simulink model "extra_tip_sim"  (Simulink 9.0)
settings: Solver=FixedStepDiscrete  StartTime=start_time  StopTime=stop_time  FixedStep=0.020  RelTol=1e-3  EnableMultiTasking=on
InitFcn:
  | extra_tip_sim_init
values from neighbouring files (symbols this model uses):
  bucketAngle = WeighDebug_TOAbucket_angle_t27    [extra_tip_sim_init.m]
  imuX = WeighDebug_TOAeef_imu_accelX_t27    [extra_tip_sim_init.m]    (also in imu_pitch_cal_sim_init.m = WeighDebug_TOAeef_imu_accelX_t194)
  imuY = WeighDebug_TOAeef_imu_accelY_t27    [extra_tip_sim_init.m]    (also in imu_pitch_cal_sim_init.m = WeighDebug_TOAeef_imu_accelY_t194)
  imuZ = WeighDebug_TOAeef_imu_accelZ_t27    [extra_tip_sim_init.m]    (also in imu_pitch_cal_sim_init.m = WeighDebug_TOAeef_imu_accelZ_t194)
  liftAngle = WeighDebug_TOAlift_angle_t27    [extra_tip_sim_init.m]    (also in imu_pitch_cal_sim_init.m = WeighDebug_TOAlift_angle_t194)
  liftCmd = WeighDebug_TOAlift_valve_cmd_t27    [extra_tip_sim_init.m]
  liftCylLength = WeighDebug_LiftCylNormLen_t27    [extra_tip_sim_init.m]    (also in imu_pitch_cal_sim_init.m = WeighDebug_LiftCylLenghtNorm_Val_t194)
  liftCylPress = WeighDebug_LiftCylPres_t27    [extra_tip_sim_init.m]    (also in imu_pitch_cal_sim_init.m = WeighDebug_LiftCylPres_t194)
  payloadTarget = TOAtestPts_toa_payload_target_final_t27    [extra_tip_sim_init.m]
  steerAng = WeighDebug_TOAsteering_angle_t27    [extra_tip_sim_init.m]    (also in imu_pitch_cal_sim_init.m = WeighDebug_TOAsteering_angle_t194)
  tiltCmd = WeighDebug_TOAtilt_valve_cmd_t27    [extra_tip_sim_init.m]
  tiltExt = WeighDebug_TOAtilt_extension_t27    [extra_tip_sim_init.m]    (also in imu_pitch_cal_sim_init.m = WeighDebug_TOAtilt_extension_t194)
  tiltHePress = WeighDebug_TOAtilt_he_pressure_t27    [extra_tip_sim_init.m]    (also in imu_pitch_cal_sim_init.m = WeighDebug_TOAtilt_he_pressure_t194)
  tiltRePress = WeighDebug_TOAtilt_re_pressure_t27    [extra_tip_sim_init.m]    (also in imu_pitch_cal_sim_init.m = WeighDebug_TOAtilt_re_pressure_t194)
  time = t27    [extra_tip_sim_init.m]    (also in imu_pitch_cal_sim_init.m = t194)
  time2 = t27    [extra_tip_sim_init.m]    (also in imu_pitch_cal_sim_init.m = t194)
  time3 = t28    [extra_tip_sim_init.m]
  toolMass = WeighDebug_TOAtool_mass_t28    [extra_tip_sim_init.m]
  unlatchTrigger = WeighDebug_TOAunlatch_trigger_t27    [extra_tip_sim_init.m]
undefined symbols (not defined in the file or in its folder): g, timestep, TipAssistLiveWeighStatus_t, TipAssistPfwStatus_t, toa_appNumber, toa_imu_lpf_cutoff_hz, toa_imuBasicOrient, toa_liftBoreDia, toa_liveLpfCutoffHz, toa_pfwLpfCutoffHz, toa_ratedPayload, toa_tiltBoreDia, toa_tiltNumCyl, toa_tiltRodDia, toa_toolBcLength
libraries: simulink x28, lib_CATutils_Utilities_ApplyName_v2 x15, lib_CATutils_Filters_1Pole_LowPass x3, tip_assist_lib x3, lib_CATutils_Timer_Countdown x3, simulink_extras x2, lib_CATutils_Override x1
(part 1 of 3)
settings Model: LogicAnalyzerSignalOrdering=a37efb6f-6706-4435-ba35-0122ce8219fd,5dd0029d-0573-49e1-b82a-316668c0f863,6142d480-2c12-41e6-bc69-adb81a4771c4,9c1653df-ca6c-4435-bc59-59c042f1a04b,d777cd1b-872a-4f45-99d0-97815b48f09e,f8fb9e00-ab92-47dd-9d0a-bc807beeb696,e773cc5f-bf5a-4589-b78e-aa1b72e66aaf,b6a03e28-23cb-43f9-a248-fda54d9653ab,b9a27f8a-7d02-4c02-ba25-8bf06c41b510,b3c5c01d-7cb6-4bb7-bbe8-a848e78f78ed,7d46beec-13ab-48f4-a3cd-fd0effd7abe8,b085631a-3729-4051-976c-78eb5fade8d3,a8a2ce2a-5a46-45c1-9d46-6a4d6193dbf9,88cdbebc-2b3c-4fe3-b108-dfac4340a4ad,5d366e23-9e16-40ab-92ec-e6241a047015,b6cb7851-fc42-42d8-ba93-f76abef1ebeb,7eca61fc-1cd1-4022-a45b-67ff63c6626d,077ebe51-704b-4e3e-9cbd-f25e18163fe1,9898f07c-b872-4868-8c48-c9d95ca54024,d8f024a4-d935-44db-a83c-243ca19a82d6,24d79649-15d2-4718-8ed2-926b01c05a24,6b01681c-0b58-4c20-ab01-5402e451f443,ac303ef7-5c28-45be-a2c5-7be4353dbcf9,456d51b4-31c5-4d8b-9e4a-36f8ba5986a5,e5bf8900-4f4f-4702-ba55-200edadc7652,7a635aaf-e9e5-4b24-8e72-5d4417a87c09,214b5661-9156-4f5f-9a6d-c54d9497f0a4,916bcfa3-db98-4ef0-9e30-7d49bd14b769,beeb6208-9be8-4a0c-9c1c-997e9a27ac07,366fba23-de5f-44fc-90b6-d2ebcc3b0ecc,6b6aee8b-916a-4cee-aecb-aa77e18be370,cc670c6b-0d83-4df0-8935-7cd51dc093c6,670c9483-bb58-4bfd-81ee-4bca25119f9a,b4fcc680-a150-49a3-beac-69dd7c97c90c,78d642a3-b1b9-4e6b-84df-a8ec2d1c8fc5,fb89492d-1250-4bf5-972c-88d3c591c784,9ec6e98f-1a7b-4b1c-b389-ae64fc96bbfa,1fbb6831-cc72-4bb8-9ab6-ce662542e337,596eca91-ee83-45ff-91c1-74049bb3a3da,0efd91b1-80a5-4fa5-9a4a-feab5d0cf49f,89142b93-7385-40ef-9b15-d3617da8d630,2ad0f06d-5e71-4340-9930-4971dfc5af72,50c9ef7d-f9c2-400a-b0a6-35ffc0f152b4,04501ed4-9feb-42f8-8fc5-352602800299,46692b40-c2fd-4c0a-8a50-25bd1b341a8a,bf056d7f-beef-4766-a4aa-f1d68af985d9,cf647fbf-2e0f-4a5b-8327-5ccd84294860,8c24ce89-e30a-461a-ac4c-7ea0b5908bdc,e7e0475a-2556-46b3-b42a-114a33c764aa,f2c2fba9-cc55-45c3-a992-41eb80094482,564b9916-4970-4188-9d93-2aecd4827002  MinMaxOverflowLogging=MinMaxAndOverflow  Creator=gulamhs  LastModifiedBy=CurriSD  SimulationMode=rapid-accelerator
settings DataIOCC: ExternalInput=[t,u]  SaveCompleteFinalSimState=on  SaveFormat=StructureWithTime  SaveOutput=off  SignalLogging=off  DSMLogging=off  SaveTime=off
settings OptimizationCC: DefaultParameterBehavior=Inlined  InlineInvariantSignals=on  EnhancedBackFolding=on  StrengthReduction=on  BitfieldContainerType=uchar_T  PassReuseOutputArgsAs=Individual arguments  ExpressionDepthLimit=2147483647  EfficientFloat2IntCast=on
settings DebuggingCC: SignalInfNanChecking=warning  SignalRangeChecking=error  ReadBeforeWriteMsg=EnableAllAsError  WriteAfterWriteMsg=EnableAllAsError  WriteAfterReadMsg=EnableAllAsError  AlgebraicLoopMsg=error  ArtificialAlgebraicLoopMsg=error  SaveWithDisabledLinksMsg=none  SaveWithParameterizedLinksMsg=error  UnderspecifiedInitializationDetection=Simplified  MergeDetectMultiDrivingBlocksExec=error  BlockPriorityViolationMsg=error  SolverPrmCheckMsg=error  InheritedTsInSrcMsg=none  TasksWithSamePriorityMsg=error  SigSpecEnsureSampleTimeMsg=error  CheckMatrixSingularityMsg=error  IntegerOverflowMsg=error  ParameterUnderflowMsg=error  ParameterPrecisionLossMsg=none  FixptConstUnderflowMsg=error  FixptConstOverflowMsg=error  UnderSpecifiedDataTypeMsg=error  FcnCallInpInsideContextMsg=warning  UnconnectedInputMsg=error  UnconnectedOutputMsg=error  UnconnectedLineMsg=error  SFcnCompatibilityMsg=error  FrameProcessingCompatibilityMsg=warning  UniqueDataStoreMsg=error  BusObjectLabelMismatch=error  RootOutportRequireBusObject=error  AssertControl=DisableAll  ModelReferenceIOMsg=error  ModelReferenceVersionMismatchMessage=warning  ModelReferenceIOMismatchMessage=error  UnknownTsInhSupMsg=error  ModelReferenceDataLoggingMessage=error  StateNameClashWarn=warning  SimStateInterfaceChecksumMismatchMsg=error  StrictBusMsg=ErrorOnBusTreatedAsVector  BusNameAdapt=ErrorWithoutRepair  NonBusSignalsTreatedAsBus=error  SFInvalidInputDataAccessInChartInitDiag=error  SFNoUnconditionalDefaultTransitionDiag=error  SFTransitionOutsideNaturalParentDiag=error  SFUnreachableExecutionPathDiag=error  SFUndirectedBroadcastEventsDiag=error  SFExecutionAtInitializationDiag=warning  IntegerSaturationMsg=error
settings HardwareCC: ProdBitPerLong=64  ProdBitPerPointer=64  ProdBitPerSizeT=64  ProdBitPerPtrDiffT=64  ProdLargestAtomicInteger=Integer  ProdLargestAtomicFloat=Float  ProdIntDivRoundTo=Zero  ProdEndianess=LittleEndian  ProdWordSize=64  ProdHWDeviceType=Intel->x86-64 (Linux 64)
settings ModelReferenceCC: ParallelModelReferenceMATLABWorkerInit=Load Top Model  PropagateSignalLabelsOutOfModel=on
settings SFSimCC: SimUserIncludeDirs=..\c_src  SFSimEcho=off  SimGenImportedTypeDefs=on  MATLABDynamicMemAlloc=off
settings SFSimCC: SimUserSources=|
  | tipoff_assist.c
  | tipoff_assist_966_14A_HL.c
  | tipoff_assist_966_14A_LOG.c
  | tipoff_assist_966_14A_STD.c
  | tipoff_assist_972_14A_HL.c
  | tipoff_assist_972_14A_STD.c
  | tipoff_assist_980_14A_HL.c
  | tipoff_assist_980_14A_STD.c
  | tipoff_assist_982_14A_LOG.c
  | tipoff_assist_982_14A_STD.c
settings RTWCC: SystemTargetFile=cat_PkgArch.tlc  GenCodeOnly=on  GenerateMakefile=off  TemplateMakefile=cat_PkgArch_default_tmf  Description=R7a CAT Package Architecture Code Generation.  GenerateReport=on  RTWUseSimCustomCode=on  CustomInclude=..\c_src  CodeProfilingSaveOptions=AllData  GenerateTraceReport=on  GenerateTraceReportSl=on  GenerateTraceReportSf=on  GenerateTraceReportEml=on  GenerateWebview=on  GenerateCodeMetricsReport=on  GenerateCodeReplacementReport=on
settings RTWCC: CustomSource=|
  | tipoff_assist.c
  | tipoff_assist_966_14A_HL.c
  | tipoff_assist_966_14A_LOG.c
  | tipoff_assist_966_14A_STD.c
  | tipoff_assist_972_14A_HL.c
  | tipoff_assist_972_14A_STD.c
  | tipoff_assist_980_14A_HL.c
  | tipoff_assist_980_14A_STD.c
  | tipoff_assist_982_14A_LOG.c
  | tipoff_assist_982_14A_STD.c
settings CodeAppCC: ForceParamTrailComments=on  IgnoreCustomStorageClasses=off  MaxIdLength=63  OperatorAnnotations=on  SimulinkDataObjDesc=on  SFDataObjDesc=on  MATLABFcnDesc=on  MangleLength=4  CustomSymbolStrType=$N$R$M  InsertBlockDesc=on  MATLABSourceComments=on  InternalIdentifier=Classic  ReqsInCode=on  UseSimReservedNames=on
settings STFCustomTargetCC: UtilityFuncGeneration=Shared location  MultiwordTypeDef=User defined  IncludeMdlTerminateFcn=off  CombineOutputUpdateFcns=on  SuppressErrorStatus=on  ERTCustomFileBanners=on  SupportAbsoluteTime=off  MultiInstanceERTCode=on  CodeInterfacePackaging=Reusable function  SupportComplex=off  SupportContinuousTime=off  SupportNonInlinedSFcns=off  RemoveResetFunc=on  SupportVariableSizeSignals=on  ParenthesesLevel=Maximum  MATLABClassNameForMDSCustomization=Simulink.SoftwareTarget.ERTCustomization  GRTInterface=off  GenerateSharedConstants=off  SystemTargetFile=cat_PkgArch.tlc
settings ERTTargetCC: UtilityFuncGeneration=Shared location  MultiwordTypeDef=User defined  MultiwordLength=2048  ParMdlRefBuildCompliant=off  CompOptLevelCompliant=off  ConcurrentExecutionCompliant=off  IncludeMdlTerminateFcn=off  SuppressErrorStatus=on  SupportAbsoluteTime=off  MultiInstanceERTCode=on  CodeInterfacePackaging=Reusable function  SupportComplex=off  SupportVariableSizeSignals=on  ParenthesesLevel=Maximum  ModelStepFunctionPrototypeControlCompliant=off  CPPClassGenCompliant=off  UseToolchainInfoCompliant=off  GenerateSharedConstants=off  MultiInstanceErrorCode=None  ERTSrcFileBannerTemplate=cat_code_template.cgt  ERTHdrFileBannerTemplate=cat_code_template.cgt  ERTDataSrcFileTemplate=cat_code_template.cgt  ERTDataHdrFileTemplate=cat_code_template.cgt  ERTCustomFileTemplate=cat_PkgArch_CFP.tlc  SuppressUnreachableDefaultCases=off  EnableUserReplacementTypes=on
settings MATStruct: int32=int32_t  int16=int16_t  int8=int8_t  uint32=uint32_t  uint16=uint16_t  uint8=uint8_t
settings CustomProperty: Value=Development
settings EnumStrPairs: String=Development
settings ConfigComp: CovScope=Subsystem  CovPath=/Chart1  CovMetricSettings=r  CovHtmlReporting=off  CovSaveCumulativeToWorkspaceVar=off  CovSaveSingleToWorkspaceVar=off  CovExternalEMLEnable=on

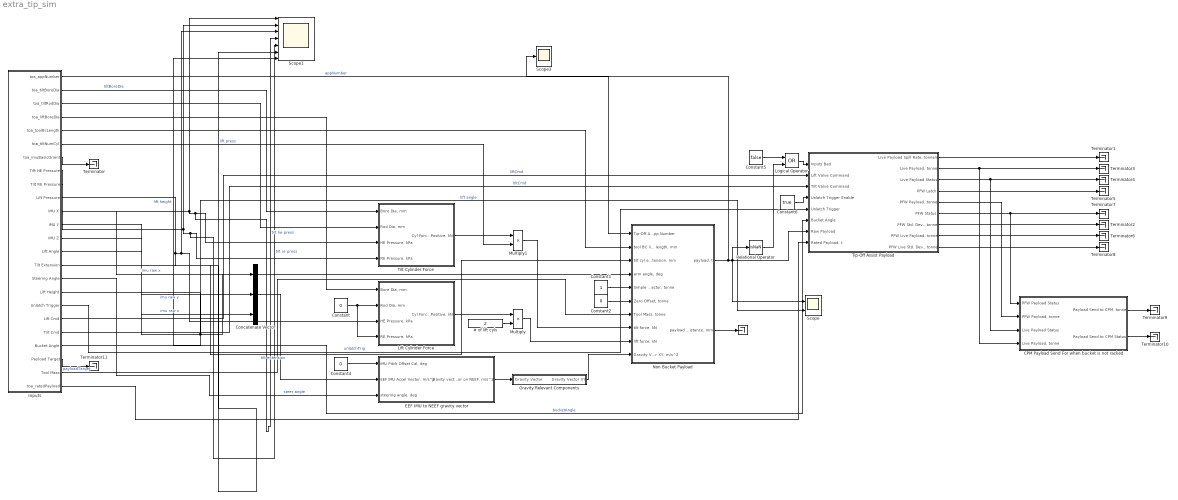
== system extra_tip_sim ==
  " " : Terminator
  # of lift cyls : Constant  Value=2  OutDataTypeStr=single
  CPM Payload Send For when bucket is not racked : Subsystem  AncestorBlock=tip_assist_lib_support/Tip-Off Assist Support Lib/CPM Payload Send For when bucket is not racked
  Concatenate Vector : Concatenate  NumInputs=3  Mode=Multidimensional array
  Constant : Constant  Value=0  OutDataTypeStr=Inherit: Inherit via back propagation
  Constant1 : Constant  OutDataTypeStr=single
  Constant2 : Constant  Value=0  OutDataTypeStr=Inherit: Inherit via back propagation
  Constant4 : Constant  Value=0  OutDataTypeStr=single
  Constant5 : Constant  Value=false  OutDataTypeStr=boolean
  Constant6 : Constant  Value=true  OutDataTypeStr=boolean
  EEF IMU to NEEF gravity vector : Subsystem
  Gravity Relevant Components : Subsystem
  "Inputs " : Subsystem
  Lift Cylinder Force : Subsystem
  Logical Operator : Logic  Operator=OR  AllPortsSameDT=off  OutDataTypeStr=boolean
  Multiply : Product  SaturateOnIntegerOverflow=on  RndMeth=Zero  InputSameDT=on  OutDataTypeStr=Inherit: Same as first input
  Multiply1 : Product  SaturateOnIntegerOverflow=on  RndMeth=Zero  InputSameDT=on  OutDataTypeStr=Inherit: Same as first input
  Non Bucket Payload : Subsystem
  Relational Operator : RelationalOperator  Operator=isNaN  OutDataTypeStr=boolean  RndMeth=Simplest
  Scope : Scope  NumInputPorts=2
  Scope1 : Scope  NumInputPorts=7
  Scope3 : Scope
  Terminator{,1..11} (12 alike) : Terminator
  Tilt Cylinder Force : Subsystem
  Tip-Off Assist Payload : Subsystem  AncestorBlock=tip_assist_lib_support/Tip-Off Assist Support Lib/Tip-Off Assist Payload
  wires:
  Multiply/1 -> Non Bucket Payload/9("lift force, kN")
  Non Bucket Payload/1("payload, t") -> Scope3/1, Tip-Off Assist Payload/7(Raw Payload), Scope/1, Relational Operator/1
  Multiply1/1 -> Non Bucket Payload/8("tilt force, kN")
  "Inputs "/6(toa_tiltNumCyl) -> Multiply1/2
  EEF IMU to NEEF gravity vector/1("gravity vector on NEEF, m/s^2") -> Gravity Relevant Components/1(Gravity Vector)
  Lift Cylinder Force/1("Cyl Force, Compression Positive, kN") -> Multiply/1
  Non Bucket Payload/2("payload distance, mm") -> " "/1
  # of lift cyls/1 -> Multiply/2
  Tilt Cylinder Force/1("Cyl Force, Compression Positive, kN") -> Multiply1/1
  Gravity Relevant Components/1(Gravity Vector XY) -> Non Bucket Payload/10("Gravity Vector XY, m/s^2")
  "Inputs "/1(toa_appNumber) -> Non Bucket Payload/1(Tip-Off Assist App Number)  "appNumber"
  "Inputs "/2(toa_tiltBoreDia) -> Tilt Cylinder Force/1("Bore Dia, mm")  "tiltBoreDia"
  "Inputs "/3(toa_tiltRodDia) -> Tilt Cylinder Force/2("Rod Dia, mm")
  "Inputs "/8(Tift HE Pressure) -> Scope1/4, Tilt Cylinder Force/3("HE Pressure, kPa"), Scope1/1  "tilt he press"
  "Inputs "/9(Tilt RE Pressure) -> Scope1/5, Tilt Cylinder Force/4("RE Pressure, kPa"), Scope1/2  "tilt re press"
  "Inputs "/4(toa_liftBoreDia) -> Lift Cylinder Force/1("Bore Dia, mm")
  "Inputs "/10(Lift Pressure) -> Scope1/6, Lift Cylinder Force/3("HE Pressure, kPa"), Scope1/3  "lift press"
  Constant/1 -> Lift Cylinder Force/4("RE Pressure, kPa"), Lift Cylinder Force/2("Rod Dia, mm")
  "Inputs "/11(IMU X) -> Concatenate Vector/1  "imu raw x"
  Concatenate Vector/1 -> EEF IMU to NEEF gravity vector/2("EEF IMU Accel Vector, m/s^2")
  "Inputs "/16(Steering Angle) -> EEF IMU to NEEF gravity vector/3("steering angle, deg")  "steer angle"
  "Inputs "/15(Tilt Extension) -> Non Bucket Payload/3("tilt cyl extension, mm")  "tilt extension"
  "Inputs "/14(Lift Angle) -> Scope/2, Non Bucket Payload/4("arm angle, deg")  "lift angle"
  "Inputs "/7(toa_imuBasicOrient) -> Terminator/1
  "Inputs "/5(toa_toolBcLength) -> Non Bucket Payload/2("tool BC link length, mm")
  Constant1/1 -> Non Bucket Payload/5("Simple Cal Factor, tonne")
  Constant2/1 -> Non Bucket Payload/6("Zero Offset, tonne")
  "Inputs "/23(Tool Mass) -> Non Bucket Payload/7("Tool Mass, tonne")
  Constant4/1 -> EEF IMU to NEEF gravity vector/1("IMU Pitch Offset Cal, deg")
  "Inputs "/17(Lift Height) -> Scope1/7  "lift height"
  "Inputs "/12(IMU Y) -> Concatenate Vector/2  "imu raw y"
  "Inputs "/13(IMU Z) -> Concatenate Vector/3  "imu raw z"
  Tip-Off Assist Payload/7("PFW Std. Dev., tonne") -> Terminator2/1
  Tip-Off Assist Payload/2("Live Payload, tonne") -> CPM Payload Send For when bucket is not racked/4("Live Payload, tonne"), Terminator3/1
  Tip-Off Assist Payload/1("Live Payload Spill Rate, tonne/s") -> Terminator1/1
  Tip-Off Assist Payload/4(PFW Latch) -> Terminator5/1
  CPM Payload Send For when bucket is not racked/1("Payload Send to CPM, tonne") -> Terminator9/1
  Tip-Off Assist Payload/9("PFW Live Std. Dev., tonne") -> Terminator8/1
  Logical Operator/1 -> Tip-Off Assist Payload/1(Inputs Bad)
  Tip-Off Assist Payload/5("PFW Payload, tonne") -> CPM Payload Send For when bucket is not racked/2("PFW Payload, tonne")
  Tip-Off Assist Payload/6(PFW Status) -> CPM Payload Send For when bucket is not racked/1(PFW Payload Status), Terminator7/1
  CPM Payload Send For when bucket is not racked/2(Payload Send to CPM Status) -> Terminator10/1
  Relational Operator/1 -> Logical Operator/2
  Tip-Off Assist Payload/3(Live Payload Status) -> CPM Payload Send For when bucket is not racked/3(Live Payload Status), Terminator4/1
  Tip-Off Assist Payload/8("PFW Live Payload, tonne") -> Terminator6/1
  Constant5/1 -> Logical Operator/1
  "Inputs "/18(Unlatch Trigger) -> Tip-Off Assist Payload/5(Unlatch Trigger)  "unlatchTrig"
  Constant6/1 -> Tip-Off Assist Payload/4(Unlatch Trigger Enable)
  "Inputs "/19(Lift Cmd) -> Tip-Off Assist Payload/2(Lift Valve Command)  "liftCmd"
  "Inputs "/20(Tilt Cmd) -> Tip-Off Assist Payload/3(Tilt Valve Command)  "tiltCmd"
  "Inputs "/21(Bucket Angle) -> Tip-Off Assist Payload/6(Bucket Angle)  "bucketAngle"
  "Inputs "/22(Payload Target) -> Terminator11/1  "payloadTarget"
  "Inputs "/24(toa_ratedPayload) -> Tip-Off Assist Payload/8("Rated Payload, t")

== system extra_tip_sim/CPM Payload Send For when bucket is not racked ==
  PFW Payload Status : Inport
  "PFW Payload, tonne" : Inport  Port=2
  Live Payload Status : Inport  Port=3
  "Live Payload, tonne" : Inport  Port=4
  MATLAB Function : MATLAB Function  TreatAsAtomicUnit=on
  "Payload Send to CPM, tonne" : Outport
  Payload Send to CPM Status : Outport  Port=2
  wires:
  MATLAB Function/2(outStatus) -> Payload Send to CPM Status/1
  MATLAB Function/1(outPayload) -> "Payload Send to CPM, tonne"/1
  Live Payload Status/1 -> MATLAB Function/3(liveStatus)
  "Live Payload, tonne"/1 -> MATLAB Function/4(livePayload)
  "PFW Payload, tonne"/1 -> MATLAB Function/2(pfwPayload)
  PFW Payload Status/1 -> MATLAB Function/1(pfwStatus)

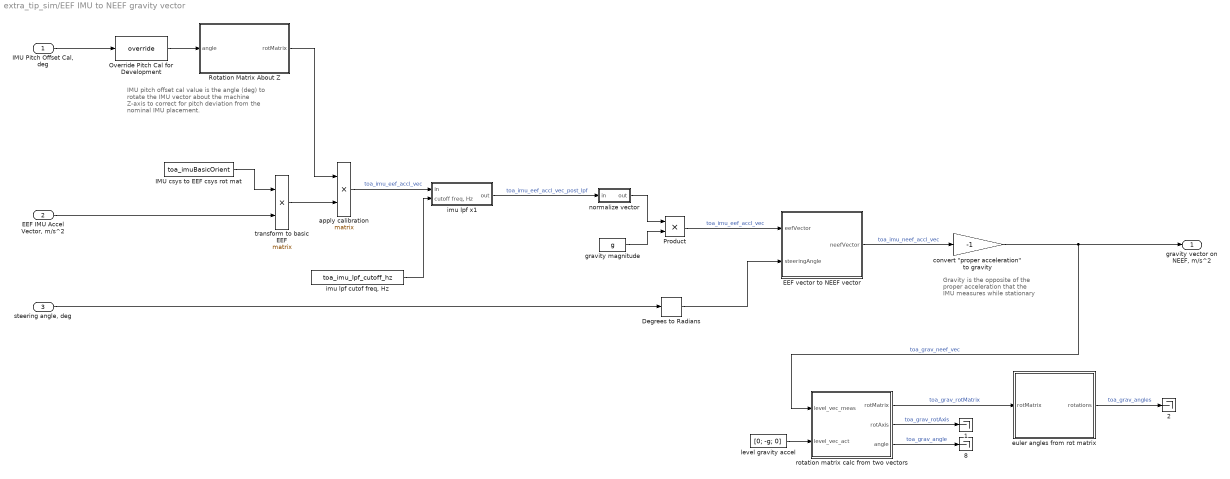
== system extra_tip_sim/EEF IMU to NEEF gravity vector ==
  note: Gravity is the opposite of the proper acceleration that the IMU measures while stationary
  note: IMU pitch offset cal value is the angle (deg) to rotate the IMU vector about the machine Z-axis to correct for pitch deviation from the nominal IMU placement.
  "IMU Pitch Offset Cal, deg" : Inport
  "EEF IMU Accel Vector, m/s^2" : Inport  Port=2
  "steering angle, deg" : Inport  Port=3
  " 1" : Terminator
  " 2" : Terminator
  " 8" : Terminator
  Degrees to Radians : simulink_extras/Transformations/Degrees to Radians
  EEF vector to NEEF vector : MATLAB Function  TreatAsAtomicUnit=on
  IMU csys to EEF csys rot mat : Constant  Value=toa_imuBasicOrient  VectorParams1D=off  OutDataTypeStr=single  SampleTime=-1
  Override Pitch Cal for Development : lib_CATutils_Override/override  ovType=OV if OV ~= Pass  extOV=off  ov_value=toa_imuCalPitchAngOv  extPass=off  pass_value=360  extRange=off  ov_max=100  ov_min=1  extCond=off  ov_cond=toa_imuCalPitchAngOv  extTF=off  ov_TrueComp=1  ov_FalseComp=2
  Product : Product  Inputs=**  OutDataTypeStr=Inherit: Same as first input
  Rotation Matrix About Z : MATLAB Function  TreatAsAtomicUnit=on
  apply calibration : Product  Multiplication=Matrix(*)  SaturateOnIntegerOverflow=on  RndMeth=Zero  OutDataTypeStr=Inherit: Same as first input
  "convert \"proper acceleration\" to gravity" : Gain  Gain=-1  SaturateOnIntegerOverflow=on  OutDataTypeStr=Inherit: Same as input  ParamDataTypeStr=Inherit: Same as input
  euler angles from rot matrix : MATLAB Function  TreatAsAtomicUnit=on
  gravity magnitude : Constant  Value=g  OutDataTypeStr=single  SampleTime=timestep
  "imu lpf cutof freq, Hz" : Constant  Value=toa_imu_lpf_cutoff_hz  OutDataTypeStr=single  SampleTime=timestep
  imu lpf x1 : Subsystem
  level gravity accel : Constant  Value=[0; -g; 0]  OutDataTypeStr=single  SampleTime=-1
  normalize vector : Subsystem
  rotation matrix calc from two vectors : MATLAB Function  TreatAsAtomicUnit=on
  transform to basic EEF : Product  Multiplication=Matrix(*)  SaturateOnIntegerOverflow=on  RndMeth=Zero  OutDataTypeStr=Inherit: Same as first input
  "gravity vector on NEEF, m/s^2" : Outport
  wires:
  "IMU Pitch Offset Cal, deg"/1 -> Override Pitch Cal for Development/1
  euler angles from rot matrix/1(rotations) -> " 2"/1  "toa_grav_angles"
  "imu lpf cutof freq, Hz"/1 -> imu lpf x1/2("cutoff freq, Hz")
  Degrees to Radians/1 -> EEF vector to NEEF vector/2(steeringAngle)
  Product/1 -> EEF vector to NEEF vector/1(eefVector)  "toa_imu_eef_accl_vec"
  "steering angle, deg"/1 -> Degrees to Radians/1
  EEF vector to NEEF vector/1(neefVector) -> "convert \"proper acceleration\" to gravity"/1  "toa_imu_neef_accl_vec"
  normalize vector/1(out) -> Product/1
  imu lpf x1/1(out) -> normalize vector/1(in)  "toa_imu_eef_accl_vec_post_lpf"
  gravity magnitude/1 -> Product/2
  Override Pitch Cal for Development/1 -> Rotation Matrix About Z/1(angle)
  Rotation Matrix About Z/1(rotMatrix) -> apply calibration/1
  apply calibration/1 -> imu lpf x1/1(in)  "toa_imu_eef_accl_vec"
  transform to basic EEF/1 -> apply calibration/2
  IMU csys to EEF csys rot mat/1 -> transform to basic EEF/1
  "convert \"proper acceleration\" to gravity"/1 -> rotation matrix calc from two vectors/1(level_vec_meas), "gravity vector on NEEF, m/s^2"/1  "toa_grav_neef_vec"
  "EEF IMU Accel Vector, m/s^2"/1 -> transform to basic EEF/2
  rotation matrix calc from two vectors/1(rotMatrix) -> euler angles from rot matrix/1(rotMatrix)  "toa_grav_rotMatrix"
  rotation matrix calc from two vectors/2(rotAxis) -> " 1"/1  "toa_grav_rotAxis"
  rotation matrix calc from two vectors/3(angle) -> " 8"/1  "toa_grav_angle"
  level gravity accel/1 -> rotation matrix calc from two vectors/2(level_vec_act)

== system extra_tip_sim/Gravity Relevant Components ==
  note: this angle is positive when the gravity vector is pointing forward in the neef XY plane
  Gravity Vector : Inport
  " neef gravity vector z" : Terminator
  " neef gravity vector z1" : Terminator
  " neef gravity vector z2" : Terminator
  Demux : Demux  Outputs=3
  Magnitude : Subsystem
  Trigonometric Function : Trigonometry  Operator=atan2  OutputSignalType=real
  Vector Concatenate1 : Concatenate  Mode=Multidimensional array
  "convert \"proper acceleration\" to gravity1" : Gain  Gain=-1  SaturateOnIntegerOverflow=on  OutDataTypeStr=Inherit: Same as input  ParamDataTypeStr=Inherit: Same as input
  Gravity Vector XY : Outport
  wires:
  Gravity Vector/1 -> Demux/1
  Demux/2 -> "convert \"proper acceleration\" to gravity1"/1, Vector Concatenate1/2
  Demux/1 -> Trigonometric Function/1, Vector Concatenate1/1
  Magnitude/1(magnitude) -> " neef gravity vector z2"/1
  Trigonometric Function/1 -> " neef gravity vector z1"/1
  "convert \"proper acceleration\" to gravity1"/1 -> Trigonometric Function/2
  Demux/3 -> " neef gravity vector z"/1
  Vector Concatenate1/1 -> Magnitude/1(vector), Gravity Vector XY/1

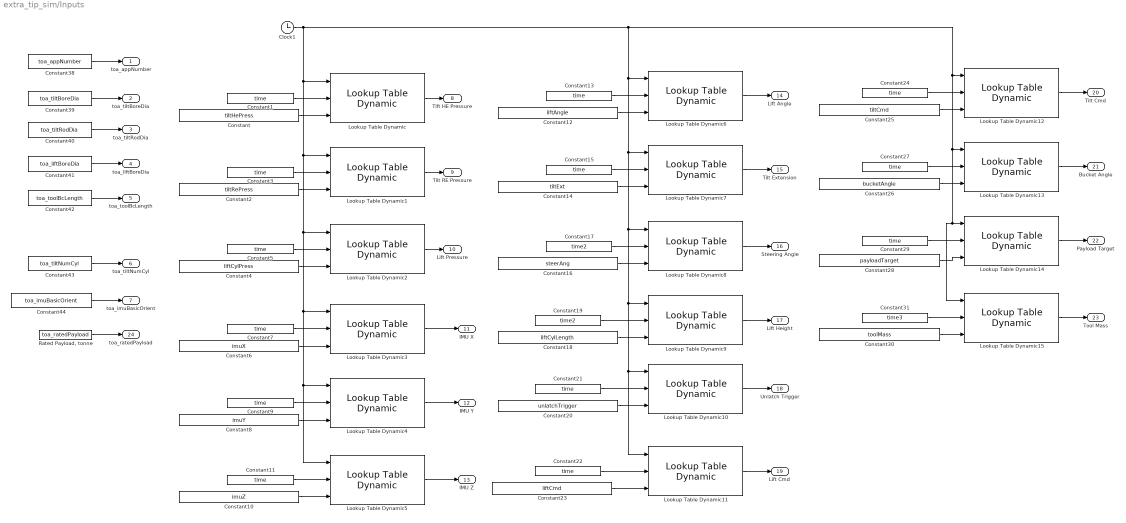
== system extra_tip_sim/Inputs  ==
  Clock1 : Clock
      settings: Decimation=1000
  Constant : Constant  Value=tiltHePress  SampleTime=timestep
  Constant{1,3,5,7,9,11,13,15,21..22,24,27,29} (13 alike) : Constant  Value=time  SampleTime=timestep
  Constant10 : Constant  Value=imuZ  SampleTime=timestep
  Constant12 : Constant  Value=liftAngle  SampleTime=timestep
  Constant14 : Constant  Value=tiltExt  SampleTime=timestep
  Constant16 : Constant  Value=steerAng  SampleTime=timestep
  Constant17 : Constant  Value=time2  SampleTime=timestep
  Constant18 : Constant  Value=liftCylLength  SampleTime=timestep
  Constant19 : Constant  Value=time2  SampleTime=timestep
  Constant2 : Constant  Value=tiltRePress  SampleTime=timestep
  Constant20 : Constant  Value=unlatchTrigger  SampleTime=timestep
  Constant23 : Constant  Value=liftCmd  SampleTime=timestep
  Constant25 : Constant  Value=tiltCmd  SampleTime=timestep
  Constant26 : Constant  Value=bucketAngle  SampleTime=timestep
  Constant28 : Constant  Value=payloadTarget  SampleTime=timestep
  Constant30 : Constant  Value=toolMass  SampleTime=timestep
  Constant31 : Constant  Value=time3  SampleTime=timestep
  Constant38 : Constant  Value=toa_appNumber  OutDataTypeStr=uint32
  Constant39 : Constant  Value=toa_tiltBoreDia  OutDataTypeStr=single
  Constant4 : Constant  Value=liftCylPress  SampleTime=timestep
  Constant40 : Constant  Value=toa_tiltRodDia  OutDataTypeStr=single
  Constant41 : Constant  Value=toa_liftBoreDia  OutDataTypeStr=single
  Constant42 : Constant  Value=toa_toolBcLength  OutDataTypeStr=single
  Constant43 : Constant  Value=toa_tiltNumCyl  OutDataTypeStr=single
  Constant44 : Constant  Value=toa_imuBasicOrient
  Constant6 : Constant  Value=imuX  SampleTime=timestep
  Constant8 : Constant  Value=imuY  SampleTime=timestep
  Lookup Table Dynamic{,1..15} (16 alike) : simulink/Lookup Tables/Lookup Table Dynamic  LookUpMeth=Interpolation-Use End Values  OutDataType=fixdt('single')  OutScaling=[]  OutputDataTypeScalingMode=Specify via dialog  OutDataTypeStr=single  DoSatur=off
      settings: SourceProductName=Simulink
  "Rated Payload, tonne" : Constant  Value=toa_ratedPayload  OutDataTypeStr=single  SampleTime=-1
  toa_appNumber : Outport  SampleTime=timestep
  toa_tiltBoreDia : Outport  Port=2  SampleTime=timestep
  toa_tiltRodDia : Outport  Port=3  SampleTime=timestep
  toa_liftBoreDia : Outport  Port=4  SampleTime=timestep
  toa_toolBcLength : Outport  Port=5  SampleTime=timestep
  toa_tiltNumCyl : Outport  Port=6  SampleTime=timestep
  toa_imuBasicOrient : Outport  Port=7  SampleTime=timestep
  Tift HE Pressure : Outport  Port=8  SampleTime=timestep
  Tilt RE Pressure : Outport  Port=9  SampleTime=timestep
  Lift Pressure : Outport  Port=10  SampleTime=timestep
  IMU X : Outport  Port=11  SampleTime=timestep
  IMU Y : Outport  Port=12  SampleTime=timestep
  IMU Z : Outport  Port=13  SampleTime=timestep
  Lift Angle : Outport  Port=14  SampleTime=timestep
  Tilt Extension : Outport  Port=15  SampleTime=timestep
  Steering Angle : Outport  Port=16  SampleTime=timestep
  Lift Height : Outport  Port=17  SampleTime=timestep
  Unlatch Trigger : Outport  Port=18  SampleTime=timestep
  Lift Cmd : Outport  Port=19  SampleTime=timestep
  Tilt Cmd : Outport  Port=20  SampleTime=timestep
  Bucket Angle : Outport  Port=21  SampleTime=timestep
  Payload Target : Outport  Port=22  SampleTime=timestep
  Tool Mass : Outport  Port=23  SampleTime=timestep
  toa_ratedPayload : Outport  Port=24  SampleTime=timestep
  wires:
  Constant17/1 -> Lookup Table Dynamic8/2
  Constant13/1 -> Lookup Table Dynamic6/2
  Lookup Table Dynamic6/1 -> Lift Angle/1
  Lookup Table Dynamic5/1 -> IMU Z/1
  Constant/1 -> Lookup Table Dynamic/3
  Lookup Table Dynamic2/1 -> Lift Pressure/1
  Constant3/1 -> Lookup Table Dynamic1/2
  Constant2/1 -> Lookup Table Dynamic1/3
  Constant8/1 -> Lookup Table Dynamic4/3
  Constant9/1 -> Lookup Table Dynamic4/2
  Constant12/1 -> Lookup Table Dynamic6/3
  Constant15/1 -> Lookup Table Dynamic7/2
  Lookup Table Dynamic7/1 -> Tilt Extension/1
  Lookup Table Dynamic8/1 -> Steering Angle/1
  Constant16/1 -> Lookup Table Dynamic8/3
  Constant11/1 -> Lookup Table Dynamic5/2
  Constant14/1 -> Lookup Table Dynamic7/3
  Constant6/1 -> Lookup Table Dynamic3/3
  Lookup Table Dynamic/1 -> Tift HE Pressure/1
  Constant4/1 -> Lookup Table Dynamic2/3
  Lookup Table Dynamic3/1 -> IMU X/1
  Lookup Table Dynamic4/1 -> IMU Y/1
  Constant1/1 -> Lookup Table Dynamic/2
  Constant7/1 -> Lookup Table Dynamic3/2
  Constant5/1 -> Lookup Table Dynamic2/2
  Constant10/1 -> Lookup Table Dynamic5/3
  Lookup Table Dynamic1/1 -> Tilt RE Pressure/1
  Constant39/1 -> toa_tiltBoreDia/1
  Constant38/1 -> toa_appNumber/1
  Constant40/1 -> toa_tiltRodDia/1
  Constant41/1 -> toa_liftBoreDia/1
  Constant42/1 -> toa_toolBcLength/1
  Constant43/1 -> toa_tiltNumCyl/1
  Constant44/1 -> toa_imuBasicOrient/1
  Clock1/1 -> Lookup Table Dynamic3/1, Lookup Table Dynamic4/1, Lookup Table Dynamic5/1, Lookup Table Dynamic2/1, Lookup Table Dynamic1/1, Lookup Table Dynamic/1, Lookup Table Dynamic14/1, Lookup Table Dynamic15/1, Lookup Table Dynamic13/1, Lookup Table Dynamic12/1, Lookup Table Dynamic8/1, Lookup Table Dynamic9/1, Lookup Table Dynamic10/1, Lookup Table Dynamic11/1, Lookup Table Dynamic7/1, Lookup Table Dynamic6/1
  Lookup Table Dynamic9/1 -> Lift Height/1
  Constant19/1 -> Lookup Table Dynamic9/2
  Constant18/1 -> Lookup Table Dynamic9/3
  Lookup Table Dynamic10/1 -> Unlatch Trigger/1
  Constant21/1 -> Lookup Table Dynamic10/2
  Constant20/1 -> Lookup Table Dynamic10/3
  Constant22/1 -> Lookup Table Dynamic11/2
  Lookup Table Dynamic11/1 -> Lift Cmd/1
  Constant23/1 -> Lookup Table Dynamic11/3
  Constant25/1 -> Lookup Table Dynamic12/3
  Lookup Table Dynamic12/1 -> Tilt Cmd/1
  Constant24/1 -> Lookup Table Dynamic12/2
  Lookup Table Dynamic13/1 -> Bucket Angle/1
  Constant26/1 -> Lookup Table Dynamic13/3
  Constant27/1 -> Lookup Table Dynamic13/2
  Lookup Table Dynamic14/1 -> Payload Target/1
  Constant29/1 -> Lookup Table Dynamic14/2
  Constant28/1 -> Lookup Table Dynamic14/3
  Constant31/1 -> Lookup Table Dynamic15/2
  Lookup Table Dynamic15/1 -> Tool Mass/1
  Constant30/1 -> Lookup Table Dynamic15/3
  "Rated Payload, tonne"/1 -> toa_ratedPayload/1

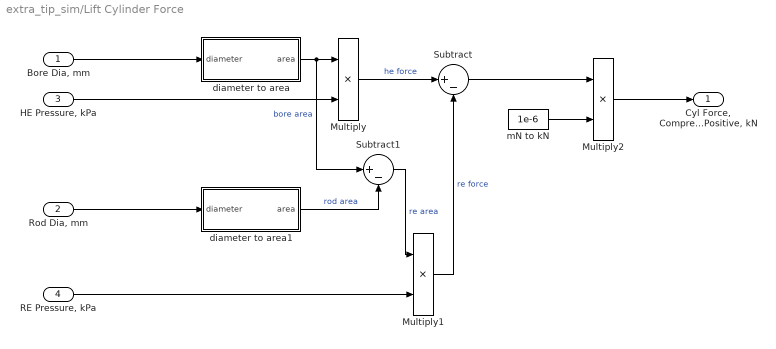
== system extra_tip_sim/Lift Cylinder Force ==
  "Bore Dia, mm" : Inport
  "Rod Dia, mm" : Inport  Port=2
  "HE Pressure, kPa" : Inport  Port=3
  "RE Pressure, kPa" : Inport  Port=4
  Multiply : Product  SaturateOnIntegerOverflow=on  RndMeth=Zero  InputSameDT=on  OutDataTypeStr=Inherit: Same as first input
  Multiply1 : Product  SaturateOnIntegerOverflow=on  RndMeth=Zero  InputSameDT=on  OutDataTypeStr=Inherit: Same as first input
  Multiply2 : Product  SaturateOnIntegerOverflow=on  RndMeth=Zero  InputSameDT=on  OutDataTypeStr=Inherit: Same as first input
  Subtract : Sum  Inputs=|+-  SaturateOnIntegerOverflow=on  InputSameDT=on  OutDataTypeStr=Inherit: Same as first input
  Subtract1 : Sum  Inputs=|+-  SaturateOnIntegerOverflow=on  InputSameDT=on  OutDataTypeStr=Inherit: Same as first input
  diameter to area : Subsystem
  diameter to area1 : Subsystem
  mN to kN : Constant  Value=1e-6  OutDataTypeStr=single
  "Cyl Force, Compression Positive, kN" : Outport
  wires:
  "HE Pressure, kPa"/1 -> Multiply/2
  Subtract/1 -> Multiply2/1
  "Bore Dia, mm"/1 -> diameter to area/1(diameter)
  Multiply1/1 -> Subtract/2  "re force"
  Multiply/1 -> Subtract/1  "he force"
  diameter to area/1(area) -> Subtract1/1, Multiply/1  "bore area"
  diameter to area1/1(area) -> Subtract1/2  "rod area"
  "RE Pressure, kPa"/1 -> Multiply1/2
  "Rod Dia, mm"/1 -> diameter to area1/1(diameter)
  Subtract1/1 -> Multiply1/1  "re area"
  mN to kN/1 -> Multiply2/2
  Multiply2/1 -> "Cyl Force, Compression Positive, kN"/1

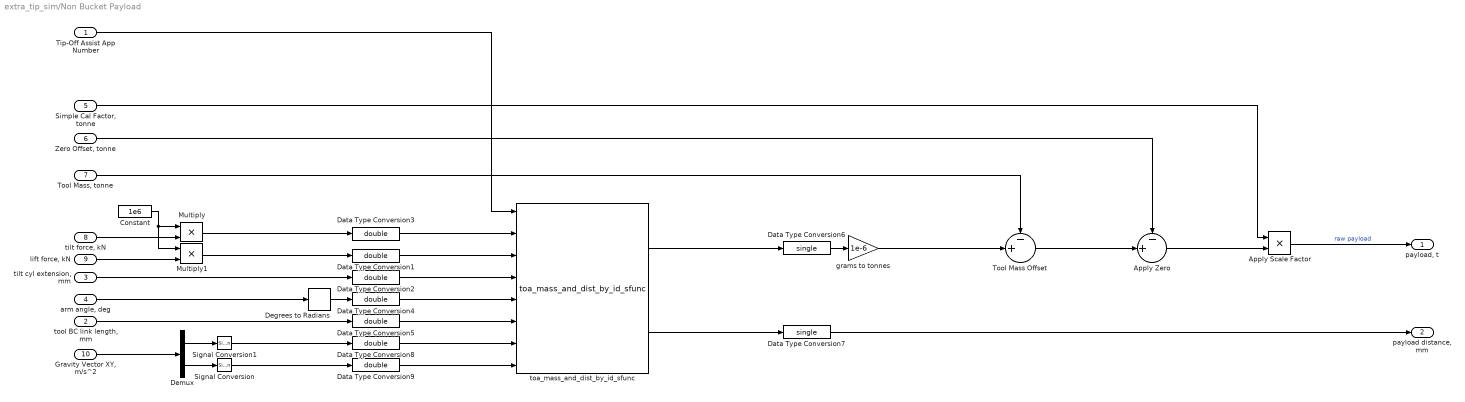
== system extra_tip_sim/Non Bucket Payload ==
  Tip-Off Assist App Number : Inport
  "tool BC link length, mm" : Inport  Port=2
  "tilt cyl extension, mm" : Inport  Port=3
  "arm angle, deg" : Inport  Port=4
  "Simple Cal Factor, tonne" : Inport  Port=5
  "Zero Offset, tonne" : Inport  Port=6
  "Tool Mass, tonne" : Inport  Port=7
  "tilt force, kN" : Inport  Port=8
  "lift force, kN" : Inport  Port=9
  "Gravity Vector XY, m/s^2" : Inport  Port=10
  Apply Scale Factor : Product
  Apply Zero : Sum  Inputs=-+|  SaturateOnIntegerOverflow=on  InputSameDT=on  OutDataTypeStr=Inherit: Same as first input
  Constant : Constant  Value=1e6  OutDataTypeStr=single
  Data Type Conversion{1..5,8..9} (7 alike) : DataTypeConversion  OutDataTypeStr=double  SaturateOnIntegerOverflow=on  RndMeth=Zero
      settings: AttributesFormatString=Output Data Type: %<OutDataTypeStr>\n
  Data Type Conversion6 : DataTypeConversion  OutDataTypeStr=single  SaturateOnIntegerOverflow=on  RndMeth=Zero
      settings: AttributesFormatString=Output Data Type: %<OutDataTypeStr>\n
  Data Type Conversion7 : DataTypeConversion  OutDataTypeStr=single  SaturateOnIntegerOverflow=on  RndMeth=Zero
      settings: AttributesFormatString=Output Data Type: %<OutDataTypeStr>\n
  Degrees to Radians : simulink_extras/Transformations/Degrees to Radians
  Demux : Demux  Outputs=2
  Multiply : Product  SaturateOnIntegerOverflow=on  RndMeth=Zero  InputSameDT=on  OutDataTypeStr=Inherit: Same as first input
  Multiply1 : Product  SaturateOnIntegerOverflow=on  RndMeth=Zero  InputSameDT=on  OutDataTypeStr=Inherit: Same as first input
  Signal Conversion : SignalConversion  OverrideOpt=on
  Signal Conversion1 : SignalConversion  OverrideOpt=on
  Tool Mass Offset : Sum  Inputs=-+|  SaturateOnIntegerOverflow=on  InputSameDT=on  OutDataTypeStr=Inherit: Same as first input
  grams to tonnes : Gain  Gain=1e-6  SaturateOnIntegerOverflow=on  OutDataTypeStr=Inherit: Same as input  ParamDataTypeStr=Inherit: Same as input
  toa_mass_and_dist_by_id_sfunc : S-Function  FunctionName=toa_mass_and_dist_by_id_sfunc  SFunctionDeploymentMode=off  EnableBusSupport=off  mask(Legacy Function){SFunctionSpec=void toa_mass_and_dist_by_id(uint32 u1, double u2, double u3, double u4, double u5, double u6, double u7, double u8, double y1[1], double y2[1]), ShowSpec=off}
      mask prompts: ShowSpec "Display function specification"
      mask help:
      | This block allows you to call the legacy functions specified by the following Legacy Code Tool definition:
      | def.SFunctionName = 'toa_mass_and_dist_by_id_sfunc';
      | def.OutputFcnSpec = 'void toa_mass_and_dist_by_id(uint32 u1, double u2, double u3, double u4, double u5, double u6, double u7, double u8, double y1[1], double y2[1])';
      | def.HeaderFiles = {'tipoff_assist.h'};
      | def.SourceFiles = {'tipoff_assist.c'};
      | def.IncPaths = {'./c_src'};
      mask Help: <p>This block was generated automatically by the Legacy Code Tool. For detailed help on this tool, call<a href="matlab:legacy_code('help')"> legacy_code('help')</a>.</p>
      mask Callback ShowSpec:
      | if strcmp(get_param(gcbh, 'ShowSpec'), 'on')
      |   set_param(gcbh, 'MaskDisplay', sprintf('fprintf(''%s'');', get_param(gcbh, 'SFunctionSpec')));
      | else
      |   set_param(gcbh, 'MaskDisplay', sprintf('fprintf(''%s'');', get_param(gcbh, 'FunctionName')));
      | end
      mask Display: fprintf('toa_mass_and_dist_by_id_sfunc');
  "payload, t" : Outport
  "payload distance, mm" : Outport  Port=2
  wires:
  Signal Conversion1/1 -> Data Type Conversion8/1
  Signal Conversion/1 -> Data Type Conversion9/1
  "tilt cyl extension, mm"/1 -> Data Type Conversion2/1
  Apply Scale Factor/1 -> "payload, t"/1  "raw payload"
  Apply Zero/1 -> Apply Scale Factor/2
  "Simple Cal Factor, tonne"/1 -> Apply Scale Factor/1
  "Zero Offset, tonne"/1 -> Apply Zero/1
  Tool Mass Offset/1 -> Apply Zero/2
  Data Type Conversion3/1 -> toa_mass_and_dist_by_id_sfunc/2
  Data Type Conversion1/1 -> toa_mass_and_dist_by_id_sfunc/3
  Data Type Conversion2/1 -> toa_mass_and_dist_by_id_sfunc/4
  Data Type Conversion4/1 -> toa_mass_and_dist_by_id_sfunc/5
  Data Type Conversion5/1 -> toa_mass_and_dist_by_id_sfunc/6
  Data Type Conversion8/1 -> toa_mass_and_dist_by_id_sfunc/7
  Data Type Conversion9/1 -> toa_mass_and_dist_by_id_sfunc/8
  Tip-Off Assist App Number/1 -> toa_mass_and_dist_by_id_sfunc/1
  "tilt force, kN"/1 -> Multiply/2
  "lift force, kN"/1 -> Multiply1/2
  Constant/1 -> Multiply1/1, Multiply/1
  Data Type Conversion6/1 -> grams to tonnes/1
  Data Type Conversion7/1 -> "payload distance, mm"/1
  "Tool Mass, tonne"/1 -> Tool Mass Offset/1
  "Gravity Vector XY, m/s^2"/1 -> Demux/1
  grams to tonnes/1 -> Tool Mass Offset/2
  toa_mass_and_dist_by_id_sfunc/2 -> Data Type Conversion7/1
  toa_mass_and_dist_by_id_sfunc/1 -> Data Type Conversion6/1
  "tool BC link length, mm"/1 -> Data Type Conversion5/1
  Demux/2 -> Signal Conversion/1
  Demux/1 -> Signal Conversion1/1
  Multiply1/1 -> Data Type Conversion1/1
  Multiply/1 -> Data Type Conversion3/1
  "arm angle, deg"/1 -> Degrees to Radians/1
  Degrees to Radians/1 -> Data Type Conversion4/1

== system extra_tip_sim/Tilt Cylinder Force ==
  "Bore Dia, mm" : Inport
  "Rod Dia, mm" : Inport  Port=2
  "HE Pressure, kPa" : Inport  Port=3
  "RE Pressure, kPa" : Inport  Port=4
  Multiply : Product  SaturateOnIntegerOverflow=on  RndMeth=Zero  InputSameDT=on  OutDataTypeStr=Inherit: Same as first input
  Multiply1 : Product  SaturateOnIntegerOverflow=on  RndMeth=Zero  InputSameDT=on  OutDataTypeStr=Inherit: Same as first input
  Multiply2 : Product  SaturateOnIntegerOverflow=on  RndMeth=Zero  InputSameDT=on  OutDataTypeStr=Inherit: Same as first input
  Subtract : Sum  Inputs=|+-  SaturateOnIntegerOverflow=on  InputSameDT=on  OutDataTypeStr=Inherit: Same as first input
  Subtract1 : Sum  Inputs=|+-  SaturateOnIntegerOverflow=on  InputSameDT=on  OutDataTypeStr=Inherit: Same as first input
  diameter to area : Subsystem
  diameter to area1 : Subsystem
  mN to kN : Constant  Value=1e-6  OutDataTypeStr=single
  "Cyl Force, Compression Positive, kN" : Outport
  wires:
  "HE Pressure, kPa"/1 -> Multiply/2
  Subtract/1 -> Multiply2/1
  "Bore Dia, mm"/1 -> diameter to area/1(diameter)
  Multiply1/1 -> Subtract/2
  Multiply/1 -> Subtract/1
  diameter to area/1(area) -> Subtract1/1, Multiply/1  "bore area"
  diameter to area1/1(area) -> Subtract1/2
  "RE Pressure, kPa"/1 -> Multiply1/2
  "Rod Dia, mm"/1 -> diameter to area1/1(diameter)
  Subtract1/1 -> Multiply1/1
  mN to kN/1 -> Multiply2/2
  Multiply2/1 -> "Cyl Force, Compression Positive, kN"/1

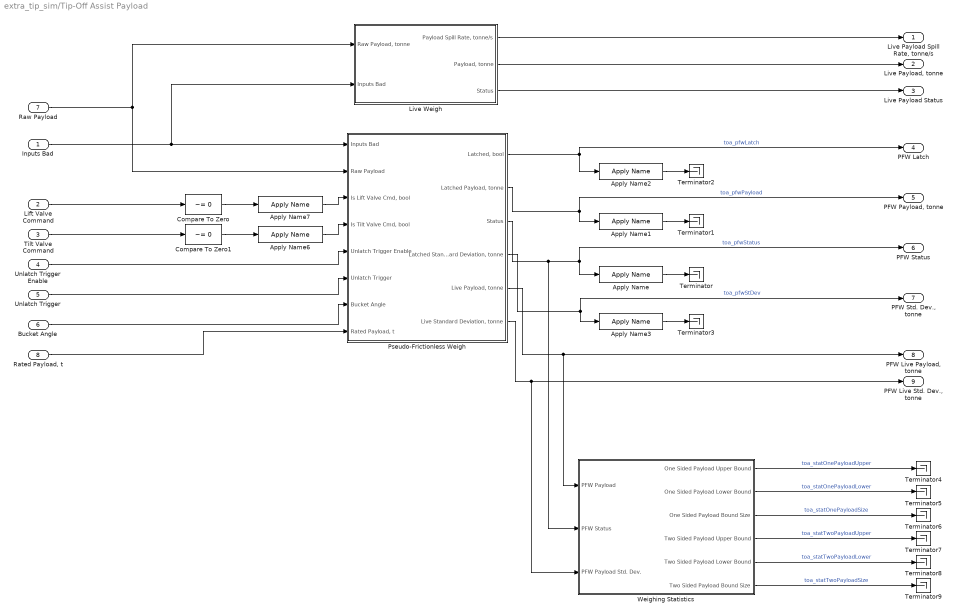
== system extra_tip_sim/Tip-Off Assist Payload ==
  Inputs Bad : Inport
  Lift Valve Command : Inport  Port=2
  Tilt Valve Command : Inport  Port=3
  Unlatch Trigger Enable : Inport  Port=4
  Unlatch Trigger : Inport  Port=5
  Bucket Angle : Inport  Port=6
  Raw Payload : Inport  Port=7
  "Rated Payload, t" : Inport  Port=8
  Apply Name : lib_CATutils_Utilities_ApplyName_v2/Apply Name  sigLabel='toa_pfwStatus2'  enTst=true
  Apply Name1 : lib_CATutils_Utilities_ApplyName_v2/Apply Name  sigLabel='toa_pfwPayload2'  enTst=true
  Apply Name2 : lib_CATutils_Utilities_ApplyName_v2/Apply Name  sigLabel='toa_pfwLatch2'  enTst=true
  Apply Name3 : lib_CATutils_Utilities_ApplyName_v2/Apply Name  sigLabel='toa_pfwStDev2'  enTst=true
  Apply Name6 : lib_CATutils_Utilities_ApplyName_v2/Apply Name  sigLabel='toa_isTiltValveCmd'  enTst=true
  Apply Name7 : lib_CATutils_Utilities_ApplyName_v2/Apply Name  sigLabel='toa_isLiftValveCmd'  enTst=true
  Compare To Zero : simulink/Logic and Bit Operations/Compare To Zero  relop=~=  OutDataTypeStr=boolean
  Compare To Zero1 : simulink/Logic and Bit Operations/Compare To Zero  relop=~=  OutDataTypeStr=boolean
  Live Weigh : Subsystem
  Pseudo-Frictionless Weigh : Subsystem
  Terminator{,1..9} (10 alike) : Terminator
  Weighing Statistics : Subsystem
  "Live Payload Spill Rate, tonne/s" : Outport
  "Live Payload, tonne" : Outport  Port=2
  Live Payload Status : Outport  Port=3
  PFW Latch : Outport  Port=4
  "PFW Payload, tonne" : Outport  Port=5
  PFW Status : Outport  Port=6
  "PFW Std. Dev., tonne" : Outport  Port=7
  "PFW Live Payload, tonne" : Outport  Port=8
  "PFW Live Std. Dev., tonne" : Outport  Port=9
  wires:
  Pseudo-Frictionless Weigh/6("Live Standard Deviation, tonne") -> Weighing Statistics/3(PFW Payload Std. Dev.), "PFW Live Std. Dev., tonne"/1
  Pseudo-Frictionless Weigh/5("Live Payload, tonne") -> Weighing Statistics/1(PFW Payload), "PFW Live Payload, tonne"/1
  Weighing Statistics/6(Two Sided Payload Bound Size) -> Terminator9/1  "toa_statTwoPayloadSize"
  Weighing Statistics/5(Two Sided Payload Lower Bound) -> Terminator8/1  "toa_statTwoPayloadLower"
  Weighing Statistics/4(Two Sided Payload Upper Bound) -> Terminator7/1  "toa_statTwoPayloadUpper"
  Weighing Statistics/3(One Sided Payload Bound Size) -> Terminator6/1  "toa_statOnePayloadSize"
  Weighing Statistics/2(One Sided Payload Lower Bound) -> Terminator5/1  "toa_statOnePayloadLower"
  Weighing Statistics/1(One Sided Payload Upper Bound) -> Terminator4/1  "toa_statOnePayloadUpper"
  Apply Name3/1 -> Terminator3/1
  Apply Name2/1 -> Terminator2/1
  Apply Name1/1 -> Terminator1/1
  Apply Name/1 -> Terminator/1
  Bucket Angle/1 -> Pseudo-Frictionless Weigh/7(Bucket Angle)
  Unlatch Trigger/1 -> Pseudo-Frictionless Weigh/6(Unlatch Trigger)
  Unlatch Trigger Enable/1 -> Pseudo-Frictionless Weigh/5(Unlatch Trigger Enable)
  Live Weigh/3(Status) -> Live Payload Status/1
  Live Weigh/2("Payload, tonne") -> "Live Payload, tonne"/1
  Live Weigh/1("Payload Spill Rate, tonne/s") -> "Live Payload Spill Rate, tonne/s"/1
  Inputs Bad/1 -> Pseudo-Frictionless Weigh/1(Inputs Bad), Live Weigh/2(Inputs Bad)
  Raw Payload/1 -> Pseudo-Frictionless Weigh/2(Raw Payload), Live Weigh/1("Raw Payload, tonne")
  Tilt Valve Command/1 -> Compare To Zero1/1
  Lift Valve Command/1 -> Compare To Zero/1
  Compare To Zero1/1 -> Apply Name6/1
  Compare To Zero/1 -> Apply Name7/1
  Pseudo-Frictionless Weigh/2("Latched Payload, tonne") -> Apply Name1/1, "PFW Payload, tonne"/1  "toa_pfwPayload"
  Pseudo-Frictionless Weigh/1("Latched, bool") -> PFW Latch/1, Apply Name2/1  "toa_pfwLatch"
  Pseudo-Frictionless Weigh/3(Status) -> Apply Name/1, PFW Status/1, Weighing Statistics/2(PFW Status)  "toa_pfwStatus"
  Pseudo-Frictionless Weigh/4("Latched Standard Deviation, tonne") -> Apply Name3/1, "PFW Std. Dev., tonne"/1  "toa_pfwStDev"
  Apply Name6/1 -> Pseudo-Frictionless Weigh/4("Is Tilt Valve Cmd, bool")
  Apply Name7/1 -> Pseudo-Frictionless Weigh/3("Is Lift Valve Cmd, bool")
  "Rated Payload, t"/1 -> Pseudo-Frictionless Weigh/8("Rated Payload, t")

== system extra_tip_sim/EEF IMU to NEEF gravity vector/imu lpf x1 ==
  in : Inport
  "cutoff freq, Hz" : Inport  Port=2
  Filter Factor Calc : Subsystem
  Single Pole Low Pass Filter : lib_CATutils_Filters_1Pole_LowPass/Single Pole Low Pass Filter  extFactor=on  extReset=off  incIntWordSize=off  mainInternalRes=off  filtFactor=.0001
  Single Pole Low Pass Filter1 : lib_CATutils_Filters_1Pole_LowPass/Single Pole Low Pass Filter  extFactor=on  extReset=off  incIntWordSize=off  mainInternalRes=off  filtFactor=.0001
  out : Outport
  wires:
  Filter Factor Calc/1(Filter Factor) -> Single Pole Low Pass Filter/2, Single Pole Low Pass Filter1/2
  "cutoff freq, Hz"/1 -> Filter Factor Calc/1(Cutoff (Hz))
  Single Pole Low Pass Filter/1 -> Single Pole Low Pass Filter1/1
  Single Pole Low Pass Filter1/1 -> out/1
  in/1 -> Single Pole Low Pass Filter/1

== system extra_tip_sim/EEF IMU to NEEF gravity vector/normalize vector ==
  in : Inport
  Divide : Product  Inputs=*/  OutDataTypeStr=Inherit: Same as first input
  Math Function : Math  Operator=square  SaturateOnIntegerOverflow=on
  Math Function1 : Math  Operator=sqrt  SaturateOnIntegerOverflow=on
  Sum of Elements : Sum  Inputs=+
  out : Outport
  wires:
  Sum of Elements/1 -> Math Function1/1
  Math Function/1 -> Sum of Elements/1
  Math Function1/1 -> Divide/2
  in/1 -> Divide/1, Math Function/1
  Divide/1 -> out/1

== system extra_tip_sim/Gravity Relevant Components/Magnitude ==
  vector : Inport
  Math Function : Math  Operator=square  SaturateOnIntegerOverflow=on
  Math Function1 : Math  Operator=sqrt  SaturateOnIntegerOverflow=on
  Sum of Elements : Sum  Inputs=+
  magnitude : Outport
  wires:
  Math Function1/1 -> magnitude/1
  Math Function/1 -> Sum of Elements/1
  Sum of Elements/1 -> Math Function1/1
  vector/1 -> Math Function/1

== system extra_tip_sim/Lift Cylinder Force/diameter to area ==
  diameter : Inport
  Constant2 : Constant  Value=pi/4  OutDataTypeStr=single
  Math Function : Math  Operator=square  OutputSignalType=real  SaturateOnIntegerOverflow=on
  Multiply2 : Product  SaturateOnIntegerOverflow=on  RndMeth=Zero  InputSameDT=on  OutDataTypeStr=Inherit: Same as first input
  area : Outport
  wires:
  Constant2/1 -> Multiply2/1
  Math Function/1 -> Multiply2/2
  Multiply2/1 -> area/1
  diameter/1 -> Math Function/1

== system extra_tip_sim/Lift Cylinder Force/diameter to area1 ==
  diameter : Inport
  Constant2 : Constant  Value=pi/4  OutDataTypeStr=single
  Math Function : Math  Operator=square  OutputSignalType=real  SaturateOnIntegerOverflow=on
  Multiply2 : Product  SaturateOnIntegerOverflow=on  RndMeth=Zero  InputSameDT=on  OutDataTypeStr=Inherit: Same as first input
  area : Outport
  wires:
  Constant2/1 -> Multiply2/1
  Math Function/1 -> Multiply2/2
  Multiply2/1 -> area/1
  diameter/1 -> Math Function/1

== system extra_tip_sim/Tilt Cylinder Force/diameter to area ==
  diameter : Inport
  Constant2 : Constant  Value=pi/4  OutDataTypeStr=single
  Math Function : Math  Operator=square  OutputSignalType=real  SaturateOnIntegerOverflow=on
  Multiply2 : Product  SaturateOnIntegerOverflow=on  RndMeth=Zero  InputSameDT=on  OutDataTypeStr=Inherit: Same as first input
  area : Outport
  wires:
  Constant2/1 -> Multiply2/1
  Math Function/1 -> Multiply2/2
  Multiply2/1 -> area/1
  diameter/1 -> Math Function/1

== system extra_tip_sim/Tilt Cylinder Force/diameter to area1 ==
  diameter : Inport
  Constant2 : Constant  Value=pi/4  OutDataTypeStr=single
  Math Function : Math  Operator=square  OutputSignalType=real  SaturateOnIntegerOverflow=on
  Multiply2 : Product  SaturateOnIntegerOverflow=on  RndMeth=Zero  InputSameDT=on  OutDataTypeStr=Inherit: Same as first input
  area : Outport
  wires:
  Constant2/1 -> Multiply2/1
  Math Function/1 -> Multiply2/2
  Multiply2/1 -> area/1
  diameter/1 -> Math Function/1
